simulink model "lab22"  (R2025b)
settings: Solver=FixedStepAuto  StartTime=0.0  StopTime=10.0  FixedStep=0.001  RelTol=1e-3
undefined symbols (not defined in the file): A, B, kappa1, kappa2, Keta, T
settings Model: Creator=Nickolay  LastModifiedBy=Nickolay

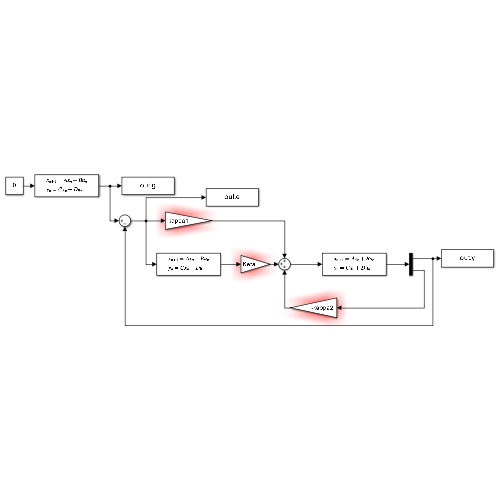
[thumbnail: Simulink's stored preview of the top-level diagram]
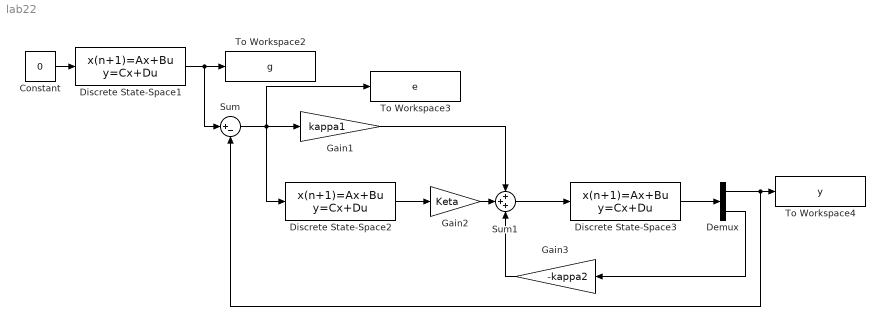
== system lab22 ==
  Constant : Constant  Value=0
  Demux : Demux  Outputs=2
  Discrete State-Space1 : DiscreteStateSpace  B=0  D=0  InitialCondition=2.8  SampleTime=T
  Discrete State-Space2 : DiscreteStateSpace  D=0  SampleTime=T
  Discrete State-Space3 : DiscreteStateSpace  A=A  B=B  C=eye(2)  D=[0; 0]  InitialCondition=[1; 0]  SampleTime=T
  Gain1 : Gain  Gain=kappa1
  Gain2 : Gain  Gain=Keta
  Gain3 : Gain  Gain=-kappa2
  Sum : Sum  Inputs=|+-
  Sum1 : Sum  Inputs=+++
  To Workspace2 : ToWorkspace  VariableName=g  SaveFormat=Timeseries  SampleTime=-1
  To Workspace3 : ToWorkspace  VariableName=e  SaveFormat=Timeseries  SampleTime=-1
  To Workspace4 : ToWorkspace  VariableName=y  SaveFormat=Timeseries  SampleTime=-1
  wires:
  Constant/1 -> Discrete State-Space1/1
  Sum/1 -> To Workspace3/1, Discrete State-Space2/1, Gain1/1
  Discrete State-Space1/1 -> Sum/1, To Workspace2/1
  Discrete State-Space2/1 -> Gain2/1
  Gain2/1 -> Sum1/2
  Gain1/1 -> Sum1/1
  Sum1/1 -> Discrete State-Space3/1
  Discrete State-Space3/1 -> Demux/1
  Demux/2 -> Gain3/1
  Gain3/1 -> Sum1/3
  Demux/1 -> To Workspace4/1, Sum/2
